simulink model "balance"  (R2025b)
settings: Solver=FixedStepDiscrete  StartTime=0.0  StopTime=10.0  FixedStep=0.1  RelTol=1e-3
values from neighbouring files (symbols this model uses):
  Offset = 16.0    [cell_balance.sldd]
settings Model: DataDictionary=cell_balance.sldd  Creator=admin  LastModifiedBy=admin
settings OptimizationCC: DefaultParameterBehavior=Inlined  EnhancedBackFolding=on  PassReuseOutputArgsAs=Individual arguments  ActiveStateOutputEnumStorageType=uint8  ZeroExternalMemoryAtStartup=off  ZeroInternalMemoryAtStartup=off  EfficientFloat2IntCast=on  OptimizeBlockOrder=speed  DifferentSizesBufferReuse=on  OptimizationCustomize=off  EfficientTunableParamExpr=on
settings DebuggingCC: ParameterTunabilityLossMsg=error
settings HardwareCC: ProdBitPerPointer=32.0  ProdBitPerSizeT=32.0  ProdBitPerPtrDiffT=32.0  ProdLargestAtomicInteger=Long  ProdLargestAtomicFloat=Double  ProdWordSize=32.0  ProdHWDeviceType=ARM Compatible->ARM Cortex-M
settings SFSimCC: MATLABDynamicMemAlloc=off
settings RTWCC: SystemTargetFile=ert.tlc  GenCodeOnly=on  TemplateMakefile=ert_default_tmf  GenerateReport=on  IncludeHyperlinkInReport=on  LaunchReport=on  GenerateTraceInfo=on  GenerateTraceReportSl=on  GenerateTraceReportSf=on  GenerateWebview=on  GPUComputeCapability=3.5  Description=Embedded Coder
settings CodeAppCC: ForceParamTrailComments=on  IgnoreCustomStorageClasses=off  OperatorAnnotations=on  SimulinkDataObjDesc=on  SFDataObjDesc=on  InsertBlockDesc=on
settings ERTTargetCC: ERTCustomFileTemplate=example_file_process.tlc  ERTFilePackagingFormat=CompactWithDataFile  DynamicArrayContainerType=coder::array  TargetLangStandard=C99 (ISO)  IncludeMdlTerminateFcn=off  SupportNonFinite=off  SupportComplex=off  RemoveDisableFunc=on

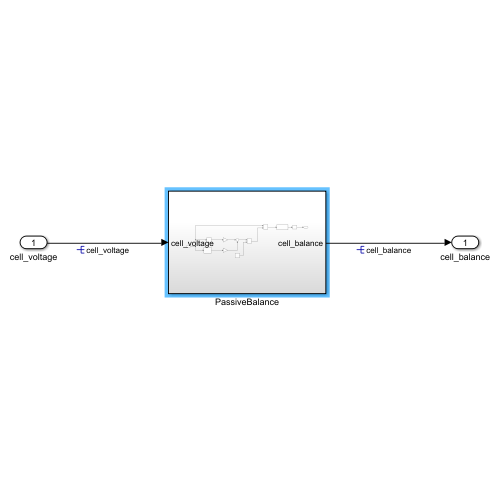
[thumbnail: Simulink's stored preview of the top-level diagram]
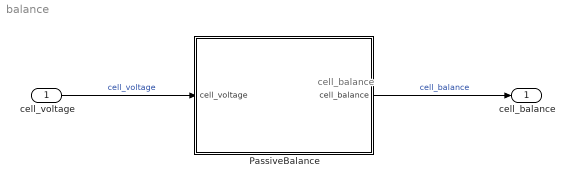
== system balance ==
  note: cell_balance
  cell_voltage : Inport
  PassiveBalance : Subsystem
  cell_balance : Outport
  wires:
  cell_voltage/1 -> PassiveBalance/1(cell_voltage)  "cell_voltage"
  PassiveBalance/1(cell_balance) -> cell_balance/1  "cell_balance"

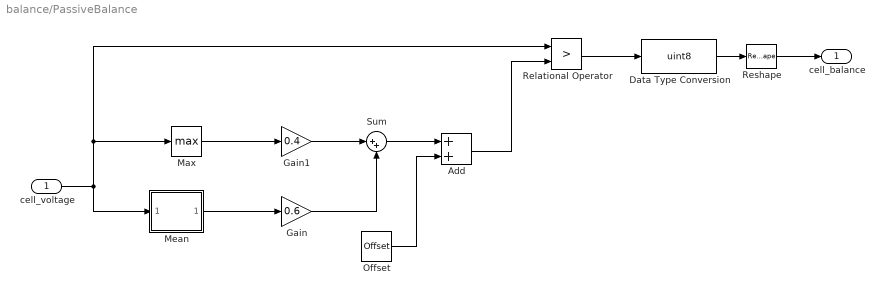
== system balance/PassiveBalance ==
  cell_voltage : Inport
  Add : Sum
  Data Type Conversion : DataTypeConversion  OutDataTypeStr=uint8  SaturateOnIntegerOverflow=off  RndMeth=Floor
  Gain : Gain  Gain=0.6
  Gain1 : Gain  Gain=0.4
  Max : MinMax  Function=max
  Mean : MATLAB Function  TreatAsAtomicUnit=on
  Offset : Constant  Value=Offset
  Relational Operator : RelationalOperator  Operator=>  OutDataTypeStr=boolean  RndMeth=Simplest  InputSameDT=off
  Reshape : Reshape  OutputDimensionality=Customize  OutputDimensions=[12,1]
  Sum : Sum  Inputs=|++
  cell_balance : Outport
  wires:
  cell_voltage/1 -> Relational Operator/1, Max/1, Mean/1(voltages)
  Sum/1 -> Add/1
  Offset/1 -> Add/2
  Gain/1 -> Sum/2
  Add/1 -> Relational Operator/2
  Max/1 -> Gain1/1
  Gain1/1 -> Sum/1
  Mean/1(avg_val) -> Gain/1
  Relational Operator/1 -> Data Type Conversion/1
  Data Type Conversion/1 -> Reshape/1
  Reshape/1 -> cell_balance/1

== matlab function balance/PassiveBalance/Mean ==
  data: voltages input; avg_val output
function avg_val = CalculateAvgIgnoringZeros(voltages)
    % 输入: voltages 是 12x1 的 uint16 列向量
    % 输出: avg_val 是 single 类型 (为了保留小数精度)
    
    sum_val = single(0); % 累加器用 single，绝对防止 uint16 溢出
    count = uint16(0);   % 计数器用 uint16 就足够了 (最多数到12)
    
    % 遍历 12 个通道
    for i = 1:length(voltages)
        % 判断电压大于 0 (uint16 只能是无符号数，不用判断小于0)
        if voltages(i) > 0
            % 将 uint16 转为 single 后累加，防止类型不匹配报错
            sum_val = sum_val + single(voltages(i)); 
            count = count + uint16(1);
        end
    end
    
    % 计算平均值，防除零保护
    if count > 0
        avg_val = sum_val / single(count); % single / single = single
    else
        avg_val = single(0);
    end
end
